simulink model "Controlled"  (R2024b)
settings: Solver=VariableStepAuto  StartTime=0.0  StopTime=s*(1/f)  RelTol=1e-9
model workspace (MAT data in the model file):
  E = 100
  L = 0.02
  R = 2
  Vpeak = 169.705627485
  alpha = 45
  f = 60
  s = 5
libraries: spsMeanLib x18, eeRmsMeasurement x18, spsCurrentMeasurementLib x9, spsVoltageMeasurementLib x9, spsACVoltageSourceLib x3, simulink x3, spsSeriesRLCBranchLib x3, spsThyristorLib x3, spsDCVoltageSourceLib x1, sps_lib x1
settings Model: Creator=Mohammed Abdelrahman  LastModifiedBy=Mohammed Abdelrahman

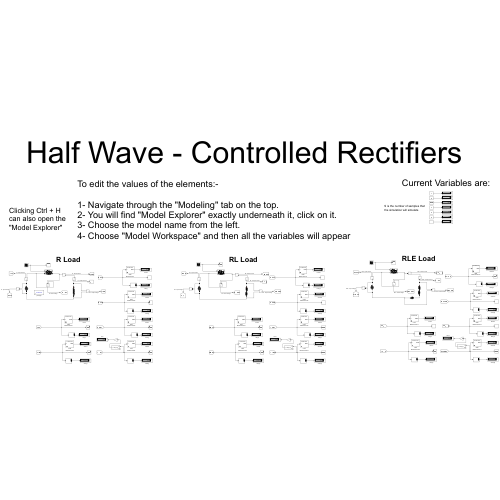
[thumbnail: Simulink's stored preview of the top-level diagram]
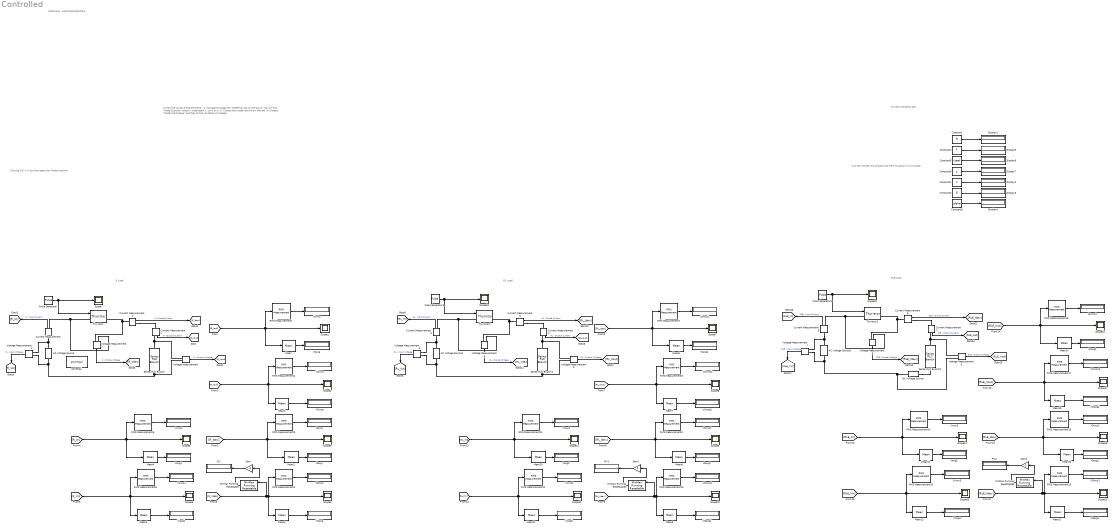
== system Controlled ==
  note: Clicking Ctrl + H can also open the "Model Explorer"
  note: S is the number of samples that the simulation will simulate
  note: Half Wave - Controlled Rectifiers
  note: To edit the values of the elements:-
      |
      | 1- Navigate through the "Modeling" tab on the top.
      | 2- You will find "Model Explorer" exactly underneath it, click on it.
      | 3- Choose the model name from the left.
      | 4- Choose "Model Workspace" and then all the variables will appear
  note: R Load
  note: RL Load
  note: RLE Load
  note: Current Variables are:
  AC Voltage Source : spsACVoltageSourceLib/AC Voltage Source  Amplitude=Vpeak  Phase=0  Frequency=f  SampleTime=0  Measurements=None  BusType=swing  Pref=10e3  Qref=0  Qmin=-inf  Qmax=+inf
  AC Voltage Source1 : spsACVoltageSourceLib/AC Voltage Source  Amplitude=Vpeak  Phase=0  Frequency=f  SampleTime=0  Measurements=None  BusType=swing  Pref=10e3  Qref=0  Qmin=-inf  Qmax=+inf
  AC Voltage Source2 : spsACVoltageSourceLib/AC Voltage Source  Amplitude=Vpeak  Phase=0  Frequency=f  SampleTime=0  Measurements=None  BusType=swing  Pref=10e3  Qref=0  Qmin=-inf  Qmax=+inf
  Constant : Constant  Value=R
  Constant1 : Constant  Value=L
  Constant2 : Constant  Value=E
  Constant3 : Constant  Value=alpha
  Constant4 : Constant  Value=f
  Constant5 : Constant  Value=Vpeak
  Constant6 : Constant  Value=s
  Current Measurement{,1..8} (9 alike) : spsCurrentMeasurementLib/Current Measurement  PhasorSimulation=off  OutputType=Complex  PSBequivalent=0
  DC Voltage Source : spsDCVoltageSourceLib/DC Voltage Source  Amplitude=E  Measurements=None
  Display{1..7} (7 alike) : Display
  Gain : Gain  Gain=-1
  Gain1 : Gain  Gain=-1
  Gain2 : Gain  Gain=-1
  IDavg : Display
  IDavg1 : Display
  IDavg2 : Display
  IDrms : Display
  IDrms1 : Display
  IDrms2 : Display
  IOavg : Display
  IOavg1 : Display
  IOavg2 : Display
  IOrms : Display
  IOrms1 : Display
  IOrms2 : Display
  Iiavg1 : Display
  Iiavg2 : Display
  Iiavg3 : Display
  Iirms1 : Display
  Iirms2 : Display
  Iirms3 : Display
  Mean{,1..17} (18 alike) : spsMeanLib/Mean  Freq=60  Vinit=0  Ts=0
  MinMax Running Resettable : simulink/Math Operations/MinMax Running Resettable  Function=min  vinit=0.0
  MinMax Running Resettable1 : simulink/Math Operations/MinMax Running Resettable  Function=min  vinit=0.0
  MinMax Running Resettable2 : simulink/Math Operations/MinMax Running Resettable  Function=min  vinit=0.0
  PIV : Display
  PIV1 : Display
  PIV2 : Display
  Pulse Generator : DiscretePulseGenerator  PulseType=Time based  Period=1/f  PulseWidth=5  PhaseDelay=alpha/(360*f)
  Pulse Generator1 : DiscretePulseGenerator  PulseType=Time based  Period=1/f  PulseWidth=5  PhaseDelay=alpha/(360*f)
  Pulse Generator2 : DiscretePulseGenerator  PulseType=Time based  Period=1/f  PulseWidth=5  PhaseDelay=alpha/(360*f)
  RMS Measurement{1..18} (18 alike) : eeRmsMeasurement/RMS Measurement  LabelModeActiveChoice=Total  F=f  SpecifyHarmonics=off  K=[0 1 2]  Ts=0
      settings: LibrarySourceBlock=|
      | ee_sl_lib/Measurements/RMS
      | Measurement
  Scope{,1..20} (21 alike) : Scope
  Series RLC Branch : spsSeriesRLCBranchLib/Series RLC Branch  LConnTagsString=__new0  RConnTagsString=__new0  BranchType=R  Resistance=R  Inductance=1e-3  SetiL0=off  InitialCurrent=0  Capacitance=1e-6  Setx0=off  InitialVoltage=0  Measurements=None
  Series RLC Branch1 : spsSeriesRLCBranchLib/Series RLC Branch  LConnTagsString=__new0  RConnTagsString=__new0  BranchType=RL  Resistance=R  Inductance=L  SetiL0=off  InitialCurrent=0  Capacitance=1e-6  Setx0=off  InitialVoltage=0  Measurements=None
  Series RLC Branch2 : spsSeriesRLCBranchLib/Series RLC Branch  LConnTagsString=__new0  RConnTagsString=__new0  BranchType=RL  Resistance=R  Inductance=L  SetiL0=off  InitialCurrent=0  Capacitance=1e-6  Setx0=off  InitialVoltage=0  Measurements=None
  Thyristor : spsThyristorLib/Thyristor  Ron=0.001  Lon=0  Vf=0.0001  IC=0  Rs=10e5  Cs=250e-9  Measurements=on
  Thyristor1 : spsThyristorLib/Thyristor  Ron=0.001  Lon=0  Vf=0.0001  IC=0  Rs=10e5  Cs=250e-9  Measurements=on
  Thyristor2 : spsThyristorLib/Thyristor  Ron=0.001  Lon=0  Vf=0.0001  IC=0  Rs=10e5  Cs=250e-9  Measurements=on
  VDavg : Display
  VDavg1 : Display
  VDavg2 : Display
  VDrms : Display
  VDrms1 : Display
  VDrms2 : Display
  VOavg : Display
  VOavg1 : Display
  VOavg2 : Display
  VOrms : Display
  VOrms1 : Display
  VOrms2 : Display
  Viavg1 : Display
  Viavg2 : Display
  Viavg3 : Display
  Virms1 : Display
  Virms2 : Display
  Virms3 : Display
  Voltage Measurement{,1..8} (9 alike) : spsVoltageMeasurementLib/Voltage Measurement  PhasorSimulation=off  OutputType=Complex  PSBequivalent=0
  powergui : sps_lib/powergui  Priority=1  SimulationMode=Continuous  SampleTime=50e-6  frequency=60  Iterations=50  frequencyindice=60  Pbase=100e6  ErrMax=1e-4  UnitsV=kV  UnitsW=MW  buscounter=0  FunctionMessages=off  echomessages=off  EnableUseOfTLC=off  CurrentSourceSwitches=off  DisableSnubberDevices=off  DisableRonSwitches=off  DisableVfSwitches=off  DisplayEquations=off  AutomaticDiscreteSolvers=off  SolverType=Tustin/Backward Euler (TBE)  Interpol=off  ExternalGateDelay=off  methode=off  Ts=100  x0status=zero  SPID=on  SwTol=0  HookPort=off  NonlinearTolerance=1e-4  nMaxIteration=100  ContinueOnMaxIteration=off  RestoreLinks=warning  ResistiveCurrentMeasurement=off  Frange=[0:2:500]  Ylog=off  Xlog=on  ShowGrid=off  save=off  variable=ZData  structure=0  ZoomFFT=off  StartTime=0.0  cycles=1  DisplayStyle=1  fundamental=60  FreqAxis=off  MaxFrequency=1000  frequencyindicesteady=1  RmsSteady=1  display=off
  wires:
  Current Measurement1/1 -> [R_Iout]  "R - Output Current"
  Voltage Measurement/1 -> [R_Vout]  "R - Output Voltage"
  Current Measurement/1 -> [R_Iin]  "R - Input Current"
  Voltage Measurement1/1 -> [R_Vin]  "R - Input Voltage"
  [R_Iout] -> Scope1/1, RMS Measurement1/1, Mean/1
  Mean1/1 -> VOavg/1
  Mean/1 -> IOavg/1
  [R_Vout] -> Mean1/1, RMS Measurement2/1, Scope2/1
  RMS Measurement2/1 -> VOrms/1
  RMS Measurement1/1 -> IOrms/1
  Voltage Measurement2/1 -> [R_Vdev]  "R - Diode Voltage"
  Current Measurement2/1 -> [R_Idev]  "R - Diode Current"
  [R_Vdev] -> RMS Measurement4/1, Scope4/1, Mean3/1, MinMax Running Resettable/1
  [R_Idev] -> Scope3/1, RMS Measurement3/1, Mean2/1
  RMS Measurement3/1 -> IDrms/1
  Mean3/1 -> VDavg/1
  Mean2/1 -> IDavg/1
  RMS Measurement4/1 -> VDrms/1
  Gain/1 -> PIV/1
  MinMax Running Resettable/1 -> Gain/1
  [R_Vin] -> Mean5/1, RMS Measurement6/1, Scope6/1
  [R_Iin] -> Scope5/1, RMS Measurement5/1, Mean4/1
  RMS Measurement5/1 -> Iirms1/1
  Mean5/1 -> Viavg1/1
  Mean4/1 -> Iiavg1/1
  RMS Measurement6/1 -> Virms1/1
  RMS Measurement12/1 -> Virms2/1
  [RL_Vout] -> Mean7/1, RMS Measurement8/1, Scope8/1
  [RL_Iout] -> Scope7/1, RMS Measurement7/1, Mean6/1
  RMS Measurement9/1 -> IDrms1/1
  RMS Measurement10/1 -> VDrms1/1
  [RL_Idev] -> Scope9/1, RMS Measurement9/1, Mean8/1
  Gain1/1 -> PIV1/1
  Mean9/1 -> VDavg1/1
  [RL_Vin] -> Mean11/1, RMS Measurement12/1, Scope12/1
  [RL_Vdev] -> RMS Measurement10/1, Scope10/1, Mean9/1, MinMax Running Resettable1/1
  RMS Measurement8/1 -> VOrms1/1
  MinMax Running Resettable1/1 -> Gain1/1
  Mean6/1 -> IOavg1/1
  Mean7/1 -> VOavg1/1
  Voltage Measurement3/1 -> [RL_Vout]  "RL - Output Voltage"
  Voltage Measurement4/1 -> [RL_Vin]  "RL - Input Voltage"
  Current Measurement3/1 -> [RL_Iin]  "RL - Input Current"
  RMS Measurement7/1 -> IOrms1/1
  RMS Measurement11/1 -> Iirms2/1
  Mean10/1 -> Iiavg2/1
  Voltage Measurement5/1 -> [RL_Vdev]  "RL - Diode Voltage"
  Mean11/1 -> Viavg2/1
  Current Measurement4/1 -> [RL_Iout]  "RL - Output Current"
  Mean8/1 -> IDavg1/1
  Current Measurement5/1 -> [RL_Idev]  "RL - Diode Current"
  [RL_Iin] -> Scope11/1, RMS Measurement11/1, Mean10/1
  Mean16/1 -> IDavg2/1
  Current Measurement7/1 -> [RLE_Iout]  "RLE - Output Current"
  [RLE_Iin] -> Scope14/1, RMS Measurement14/1, Mean12/1
  Mean14/1 -> IOavg2/1
  Mean13/1 -> Viavg3/1
  Voltage Measurement8/1 -> [RLE_Vdev]  "RLE - Diode Voltage"
  Voltage Measurement7/1 -> [RLE_Vin]  "RLE - Input Voltage"
  Current Measurement8/1 -> [RLE_Idev]  "RLE - Diode Current"
  Mean12/1 -> Iiavg3/1
  RMS Measurement14/1 -> Iirms3/1
  Voltage Measurement6/1 -> [RLE_Vout]  "RLE - Output Voltage"
  [RLE_Vin] -> Mean13/1, RMS Measurement15/1, Scope15/1
  Mean15/1 -> VOavg2/1
  Gain2/1 -> PIV2/1
  [RLE_Vdev] -> RMS Measurement13/1, Scope13/1, Mean17/1, MinMax Running Resettable2/1
  MinMax Running Resettable2/1 -> Gain2/1
  Mean17/1 -> VDavg2/1
  [RLE_Idev] -> Scope18/1, RMS Measurement18/1, Mean16/1
  RMS Measurement17/1 -> VOrms2/1
  RMS Measurement15/1 -> Virms3/1
  RMS Measurement18/1 -> IDrms2/1
  [RLE_Iout] -> Scope16/1, RMS Measurement16/1, Mean14/1
  Current Measurement6/1 -> [RLE_Iin]  "RLE - Input Current"
  [RLE_Vout] -> Mean15/1, RMS Measurement17/1, Scope17/1
  RMS Measurement13/1 -> VDrms2/1
  RMS Measurement16/1 -> IOrms2/1
  Constant5/1 -> Display6/1
  Constant/1 -> Display1/1
  Constant6/1 -> Display7/1
  Constant1/1 -> Display2/1
  Constant4/1 -> Display5/1
  Constant2/1 -> Display3/1
  Pulse Generator/1 -> Thyristor/1, Scope/1
  Constant3/1 -> Display4/1
  Pulse Generator1/1 -> Thyristor1/1, Scope19/1
  Pulse Generator2/1 -> Thyristor2/1, Scope20/1
  connections:
  Current Measurement/LConn1 -- Voltage Measurement1/LConn2 -- AC Voltage Source/RConn1
  Current Measurement/RConn1 -- Thyristor/LConn1 -- Voltage Measurement2/LConn1
  Series RLC Branch/LConn1 -- Voltage Measurement/LConn1 -- Current Measurement1/RConn1
  Series RLC Branch/RConn1 -- Voltage Measurement/LConn2 -- Voltage Measurement1/LConn1 -- AC Voltage Source/LConn1
  Voltage Measurement2/LConn2 -- Thyristor/RConn1 -- Current Measurement2/LConn1
  Current Measurement2/RConn1 -- Current Measurement1/LConn1
  Current Measurement3/LConn1 -- Voltage Measurement4/LConn2 -- AC Voltage Source1/RConn1
  AC Voltage Source1/LConn1 -- Series RLC Branch1/RConn1 -- Voltage Measurement3/LConn2 -- Voltage Measurement4/LConn1
  Current Measurement5/LConn1 -- Thyristor1/RConn1 -- Voltage Measurement5/LConn2
  Current Measurement3/RConn1 -- Thyristor1/LConn1 -- Voltage Measurement5/LConn1
  Voltage Measurement3/LConn1 -- Series RLC Branch1/LConn1 -- Current Measurement4/RConn1
  Current Measurement5/RConn1 -- Current Measurement4/LConn1
  Current Measurement6/RConn1 -- Thyristor2/LConn1 -- Voltage Measurement8/LConn1
  Voltage Measurement6/LConn2 -- DC Voltage Source/LConn1 -- Voltage Measurement7/LConn1 -- AC Voltage Source2/LConn1
  Current Measurement8/LConn1 -- Thyristor2/RConn1 -- Voltage Measurement8/LConn2
  Current Measurement6/LConn1 -- Voltage Measurement7/LConn2 -- AC Voltage Source2/RConn1
  Voltage Measurement6/LConn1 -- Series RLC Branch2/LConn1 -- Current Measurement7/RConn1
  Current Measurement8/RConn1 -- Current Measurement7/LConn1
  DC Voltage Source/RConn1 -- Series RLC Branch2/RConn1
